simulink model "aero2_position_control_experiment"  (R2024b)
settings: Solver=ode1  StartTime=0.0  StopTime=60  FixedStep=0.002  RelTol=1e-3
model workspace (MAT data in the model file):
  Dq = 3.88928113461
  Kff = 1
  Kq = 3.78162693601
  Reference = [0 0.002 0.004 0.006 0.008 0.01 0.012 0.014 0.016 0.018 0.02 0.022 ... (90003 elements, 30001x3)]
  ReferenceRate = [0 0.002 0.004 0.006 0.008 0.01 0.012 0.014 0.016 0.018 0.02 0.022 ... (90003 elements, 30001x3)]
  U_h = timeseries
  U_h.Name = 'unnamed'
  U_h.DataInfo = tsdata.datametadata
  U_h.DataInfo.Interpolation = tsdata.interpolation
  U_h.DataInfo.Interpolation.Fhandle : function handle (value not decoded)
  U_h.DataInfo.Interpolation.Name = 'linear'
  U_h.TimeInfo = tsdata.timemetadata
  U_h.TimeInfo.Length = 30001
  U_h.TimeInfo.DuplicateTimes = 0
  U_h.TimeInfo.Time_ = [0 0.002 0.004 0.006 0.008 0.01 0.012 0.014 0.016 0.018 0.02 0.022 ... (30001 elements, 30001x1)]
  U_h.TimeInfo.Initialized = 1
  U_h.QualityInfo = tsdata.qualmetadata
  U_h.Data_ = [0 0 0 0 0 0 0 0 0 0 0 0 ... (30001 elements, 30001x1)]
  U_v = timeseries
  U_v.Name = 'unnamed'
  U_v.DataInfo = tsdata.datametadata
  U_v.DataInfo.Interpolation = tsdata.interpolation
  U_v.DataInfo.Interpolation.Fhandle : function handle (value not decoded)
  U_v.DataInfo.Interpolation.Name = 'linear'
  U_v.TimeInfo = tsdata.timemetadata
  U_v.TimeInfo.Length = 30001
  U_v.TimeInfo.DuplicateTimes = 0
  U_v.TimeInfo.Time_ = [0 0.002 0.004 0.006 0.008 0.01 0.012 0.014 0.016 0.018 0.02 0.022 ... (30001 elements, 30001x1)]
  U_v.TimeInfo.Initialized = 1
  U_v.QualityInfo = tsdata.qualmetadata
  U_v.Data_ = [0 0 0 0 0 0 0 0 0 0 0 0 ... (30001 elements, 30001x1)]
  X0 = [0; 0; 0; 0]
(part 1 of 2)
settings Model: Creator=matiasgarcia  LastModifiedBy=matiasgarcia
settings DataIOCC: SaveOutput=off  SignalLogging=off  SaveTime=off

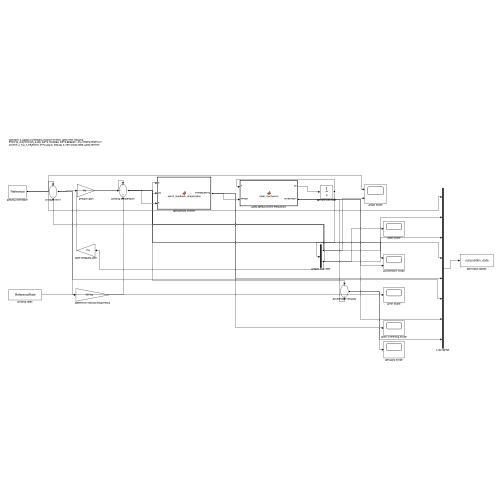
[thumbnail: Simulink's stored preview of the top-level diagram]
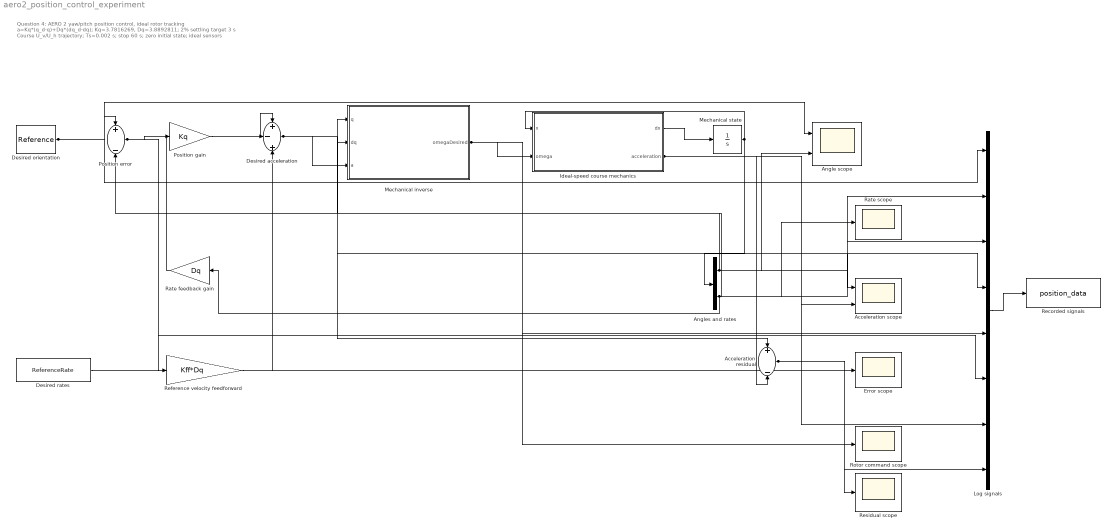
== system aero2_position_control_experiment ==
  note: Question 4: AERO 2 yaw/pitch position control, ideal rotor tracking
      | a=Kq*(q_d-q)+Dq*(dq_d-dq); Kq=3.7816269, Dq=3.8892811; 2% settling target 3 s
      | Course U_v/U_h trajectory; Ts=0.002 s; stop 60 s; zero initial state; ideal sensors
  Acceleration residual : Sum  Inputs=+-
  Acceleration scope : Scope  NumInputPorts=2
  Angle scope : Scope  NumInputPorts=2
  Angles and rates : Demux  Outputs=[2 2]
  Desired acceleration : Sum  Inputs=+-+
  Desired orientation : FromWorkspace  VariableName=Reference  OutputAfterFinalValue=Holding final value
  Desired rates : FromWorkspace  VariableName=ReferenceRate  OutputAfterFinalValue=Holding final value
  Error scope : Scope
  Ideal-speed course mechanics : MATLAB Function  TreatAsAtomicUnit=on
  Log signals : Mux  Inputs=8
  Mechanical inverse : MATLAB Function  TreatAsAtomicUnit=on
  Mechanical state : Integrator  InitialCondition=X0
  Position error : Sum  Inputs=+-
  Position gain : Gain  Gain=Kq
  Rate feedback gain : Gain  Gain=Dq
  Rate scope : Scope
  Recorded signals : ToWorkspace  VariableName=position_data  SaveFormat=Timeseries  SampleTime=-1
  Reference velocity feedforward : Gain  Gain=Kff*Dq
  Residual scope : Scope
  Rotor command scope : Scope
  wires:
  Angles and rates/1 -> Position error/2, Mechanical inverse/1(q), Angle scope/2, Log signals/2
  Position error/1 -> Position gain/1, Error scope/1, Log signals/6
  Position gain/1 -> Desired acceleration/1
  Angles and rates/2 -> Rate feedback gain/1, Mechanical inverse/2(dq), Rate scope/1, Log signals/3
  Rate feedback gain/1 -> Desired acceleration/2
  Desired acceleration/1 -> Mechanical inverse/3(a), Acceleration scope/1, Acceleration residual/1, Log signals/4
  Mechanical inverse/1(omegaDesired) -> Ideal-speed course mechanics/2(omega), Rotor command scope/1, Log signals/5
  Mechanical state/1 -> Ideal-speed course mechanics/1(x), Angles and rates/1
  Ideal-speed course mechanics/1(dx) -> Mechanical state/1
  Ideal-speed course mechanics/2(acceleration) -> Acceleration scope/2, Acceleration residual/2, Log signals/7
  Desired rates/1 -> Reference velocity feedforward/1
  Reference velocity feedforward/1 -> Desired acceleration/3
  Acceleration residual/1 -> Residual scope/1, Log signals/8
  Log signals/1 -> Recorded signals/1
  Desired orientation/1 -> Position error/1, Angle scope/1, Log signals/1
